simulink model "NBMS_Regen"  (R2026b)
settings: Solver=FixedStepDiscrete  StopTime=25  FixedStep=0.1
undefined symbols (not defined in the file): BMS_MODE_E, X_RCL_CONT_SAFETY_PACK, Y_RCL_CONT_SAFETY_PACK
libraries: simulink x1
settings Model: Creator=dell  LastModifiedBy=rathi
settings OptimizationCC: DefaultParameterBehavior=Inlined  DifferentSizesBufferReuse=on  EfficientTunableParamExpr=on  EnhancedBackFolding=on  OptimizationCustomize=off  OptimizeBlockOrder=speed  PassReuseOutputArgsAs=Individual arguments  RemoveInternalMemoryZeroInit=on  RemoveRootLevelIOMemoryZeroInit=on
settings DebuggingCC: ParameterTunabilityLossMsg=error
settings SFSimCC: MATLABDynamicMemAlloc=off
settings RTWCC: Description=Embedded Coder  GenCodeOnly=on  PackageGeneratedCodeAndArtifacts=on  SystemTargetFile=ert.tlc  TemplateMakefile=ert_default_tmf
settings CodeAppCC: ForceParamTrailComments=on  IgnoreCustomStorageClasses=off  InsertBlockDesc=on  OperatorAnnotations=on  SFDataObjDesc=on  SimulinkDataObjDesc=on
settings ERTTargetCC: DynamicArrayContainerType=coder::array  GenerateSampleERTMain=on
settings ConfigComp: DVDefectChecker=on  DVDetectOutOfBounds=on  DVHarnessSource=Signal Editor  DVModelReferenceHarness=on  DVTestSuiteOptimization=Auto

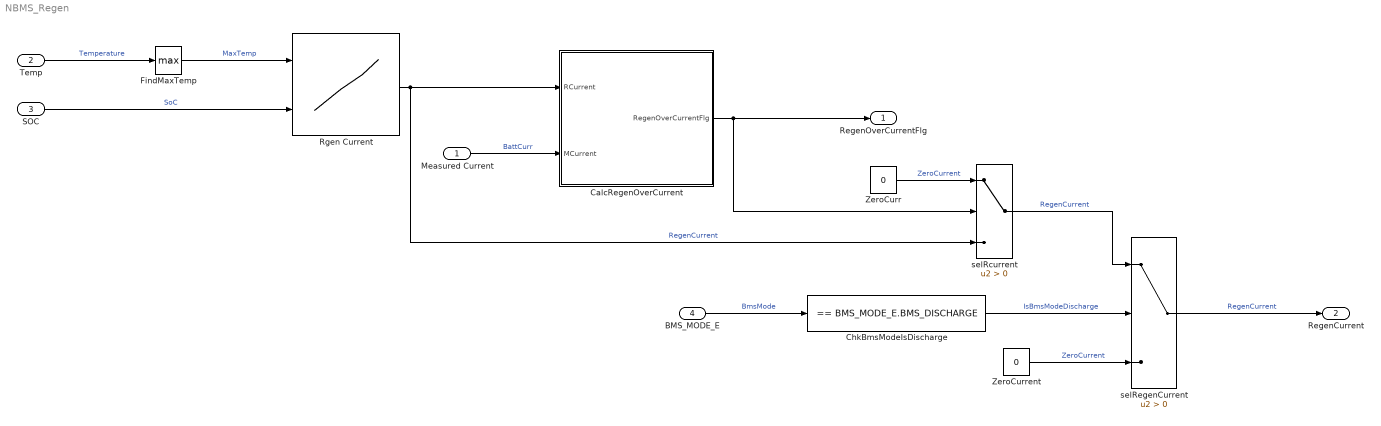
== system NBMS_Regen ==
  Measured Current : Inport  OutDataTypeStr=double
  Temp : Inport  Port=2  OutDataTypeStr=double  PortDimensions=[6,1]
  SOC : Inport  Port=3  OutDataTypeStr=double
  BMS_MODE_E : Inport  Port=4  OutDataTypeStr=Enum: BMS_MODE_E
  CalcRegenOverCurrent : Stateflow chart  TreatAsAtomicUnit=on
      settings: PortSchema="{\"entries\":[{\"content\":{\"sides\":[{\"content\":{\"connectorIds\":[\"In2\",\"In1\"]},\"type\":\"ConnectorPlacement.EquallySpacedRectSide\",\"uuid\":\"52bb604b-909c-4c3e-bef6-ce1d1f5054da\"},{\"content\":{\"connectorIds\":[\"Out1\"],\"side\":\"RIGHT\"},\"type\":\"ConnectorPlacement.EquallySpacedRectSide\",\"uuid\":\"d38b8461-b4d5-4160-a6f6-fadb19e41a68\"},{\"content\":{\"side\":\"TOP\"},\"type\":\"ConnectorPlacement.EquallySpacedRectSide\",\"uuid\":\"00e1da94-be57-4431-89b6-445e2e44a3a0\"},{\"content\":{\"side\":\"BOTTOM\"},\"type\":\"ConnectorPlacement.EquallySpacedRectSide\",\"uuid\":\"da6919b0-07bf-4ffb-a587-1cfb3b9835bc\"}]},\"type\":\"ConnectorPlacement.EquallySpacedConnector\",\"uuid\":\"263c8d4f-6461-4729-ab0c-0e10d7c24bb2\"}],\"packageUris\":[\"http://schema.mathworks.com/mf0/Connector/R2020b\"],\"version\":\"1.0\"}"
  ChkBmsModeIsDischarge : simulink/Logic and Bit Operations/Compare To Constant  relop===  const=BMS_MODE_E.BMS_DISCHARGE  OutDataTypeStr=boolean
  FindMaxTemp : MinMax  Function=max
  Rgen Current : Lookup_n-D  BreakpointsForDimension1=X_RCL_CONT_SAFETY_PACK  BreakpointsForDimension2=Y_RCL_CONT_SAFETY_PACK  BreakpointsForDimension1DataTypeStr=Inherit: Inherit from 'Breakpoint data'  BreakpointsForDimension2DataTypeStr=Inherit: Inherit from 'Breakpoint data'  Table=[0 0 0 0 0 0 0 0 0 0 0 0 0; 0 0 0 0 0 0 0 0 0 0 0 0 0; 0 0 0 0 0 0 0 0 0 0 0 0 0; 52 52 52 52 52 52 52 49 35 21 14 7 0; 52 52 52 52 52 52 52 52 49 35 21 17 2; 52 52 52 52 52 52 52 52 52 49 28 21 2; 52 52 52 52 52 52 52 52 52 49 28 21 2; 52 52 52 52 52 52 52 52 52 49 28 21 2; 0 0 0 0 0 0 0 0 0 0 0 0 0];  InternalRulePriority=Speed  RndMeth=Simplest
      settings: InputPortMap=u0,u1
  ZeroCurr : Constant  Value=0
  ZeroCurrent : Constant  Value=0  OutDataTypeStr=Inherit: Inherit via back propagation
  selRcurrent : Switch  Criteria=u2 > Threshold  SaturateOnIntegerOverflow=off  InputSameDT=off
  selRegenCurrent : Switch  Criteria=u2 > Threshold  SaturateOnIntegerOverflow=off  InputSameDT=off
  RegenOverCurrentFlg : Outport  OutDataTypeStr=boolean
  RegenCurrent : Outport  Port=2  OutDataTypeStr=double
  wires:
  BMS_MODE_E/1 -> ChkBmsModeIsDischarge/1  "BmsMode"
  Temp/1 -> FindMaxTemp/1  "Temperature"
  FindMaxTemp/1 -> Rgen Current/1  "MaxTemp"
  CalcRegenOverCurrent/1(RegenOverCurrentFlg) -> RegenOverCurrentFlg/1, selRcurrent/2
  Measured Current/1 -> CalcRegenOverCurrent/1(MCurrent)  "BattCurr"
  Rgen Current/1 -> selRcurrent/3, CalcRegenOverCurrent/2(RCurrent)  "RegenCurrent"
  ZeroCurr/1 -> selRcurrent/1  "ZeroCurrent"
  selRcurrent/1 -> selRegenCurrent/1  "RegenCurrent"
  ChkBmsModeIsDischarge/1 -> selRegenCurrent/2  "IsBmsModeDischarge"
  ZeroCurrent/1 -> selRegenCurrent/3  "ZeroCurrent"
  selRegenCurrent/1 -> RegenCurrent/1  "RegenCurrent"
  SOC/1 -> Rgen Current/2  "SoC"

== stateflow chart NBMS_Regen/CalcRegenOverCurrent ==
  state Comparison
    en,du:
    RegenOverCurrentFlg=boolean(0);
  state result
    en,du:
    RegenOverCurrentFlg=boolean(1);
  (default) -> Comparison
  result -> Comparison : [duration (MCurrent < RCurrent) > RegenAllowedTime]
  Comparison -> result : [duration (MCurrent > RCurrent) > RegenAllowedTime]
  data: MCurrent input; RCurrent input; RegenAllowedTime parameter; RegenOverCurrentFlg output
